simulink model "cst_planning"  (R2023a)
settings: configuration reference "config" (kept outside this file)
undefined symbols (not defined in the file): DiscIntNeverNeededParam
settings Model: DataDictionary=model_config.sldd  Creator=huangcheng  LastModifiedBy=Administrator
settings ConfigSetRef: SourceName=config

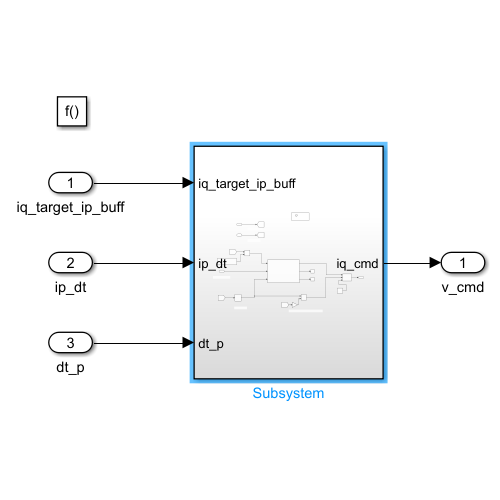
[thumbnail: Simulink's stored preview of the top-level diagram]
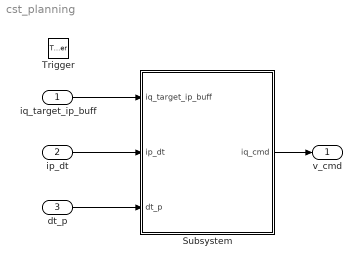
== system cst_planning ==
  iq_target_ip_buff : Inport  OutDataTypeStr=single  PortDimensions=4
  ip_dt : Inport  Port=2
  dt_p : Inport  Port=3
  Trigger : TriggerPort  TriggerType=function-call  VariantControl=(inherit)  PortDimensions=1
  Subsystem : Subsystem
  v_cmd : Outport
  wires:
  iq_target_ip_buff/1 -> Subsystem/1(iq_target_ip_buff)
  ip_dt/1 -> Subsystem/2(ip_dt)
  Subsystem/1(iq_cmd) -> v_cmd/1
  dt_p/1 -> Subsystem/3(dt_p)

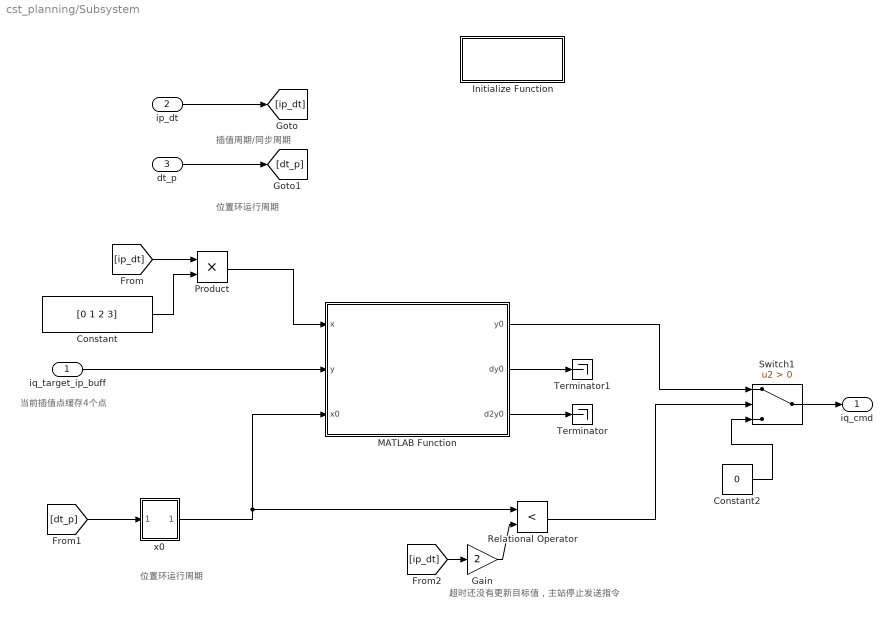
== system cst_planning/Subsystem ==
  note: 插值周期/同步周期
  note: 位置环运行周期
  note: 当前插值点缓存4个点
  note: 位置环运行周期
  note: 超时还没有更新目标值，主站停止发送指令
  iq_target_ip_buff : Inport  OutDataTypeStr=single  PortDimensions=4
  ip_dt : Inport  Port=2
  dt_p : Inport  Port=3
  Constant : Constant  Value=[0 1 2 3]  OutDataTypeStr=single
  Constant2 : Constant  Value=0  OutDataTypeStr=single
  Gain : Gain  Gain=2
  Initialize Function : Subsystem  TreatAsAtomicUnit=on
  MATLAB Function : MATLAB Function  SystemSampleTime=10e-5
  Product : Product
  Relational Operator : RelationalOperator  Operator=<  OutDataTypeStr=boolean  RndMeth=Simplest  InputSameDT=off
  Switch1 : Switch  Criteria=u2 > Threshold  SaturateOnIntegerOverflow=off  InputSameDT=off
  Terminator : Terminator
  Terminator1 : Terminator
  x0 : Subsystem
  iq_cmd : Outport
  wires:
  dt_p/1 -> [dt_p]
  ip_dt/1 -> [ip_dt]
  iq_target_ip_buff/1 -> MATLAB Function/2(y)
  Constant/1 -> Product/2
  MATLAB Function/3(d2y0) -> Terminator/1
  Product/1 -> MATLAB Function/1(x)
  [ip_dt] -> Product/1
  MATLAB Function/2(dy0) -> Terminator1/1
  [dt_p] -> x0/1(In1)
  [ip_dt] -> Gain/1
  Gain/1 -> Relational Operator/2
  Relational Operator/1 -> Switch1/2
  x0/1(x0) -> Relational Operator/1, MATLAB Function/3(x0)
  Constant2/1 -> Switch1/3
  Switch1/1 -> iq_cmd/1
  MATLAB Function/1(y0) -> Switch1/1

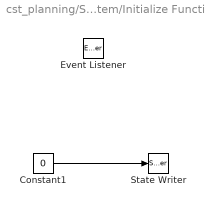
== system cst_planning/Subsystem/Initialize Function ==
  Constant1 : Constant  Value=0  OutDataTypeStr=single
  Event Listener : EventListener  DisableCoverage=on  EventName=reset
  State Writer : StateWriter  StateOwnerBlock=../../x0/Discrete-Time Integrator  StateName=x0_sum
  wires:
  Constant1/1 -> State Writer/1

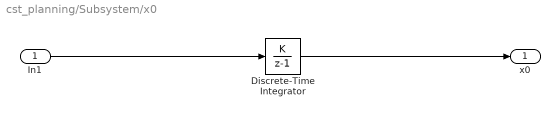
== system cst_planning/Subsystem/x0 ==
  In1 : Inport
  Discrete-Time Integrator : DiscreteIntegrator  IntegratorMethod=Accumulation: Forward Euler  SampleTime=-1  StateName=x0_sum  ICPrevOutput=DiscIntNeverNeededParam  ICPrevScaledInput=DiscIntNeverNeededParam
  x0 : Outport
  wires:
  In1/1 -> Discrete-Time Integrator/1
  Discrete-Time Integrator/1 -> x0/1

== matlab function cst_planning/Subsystem/MATLAB Function ==
  data: x input; y input; y0 output; x0 input; dy0 output; d2y0 output
function [y0, dy0, d2y0]  = InterpolateSignal(x,y,x0)
 
 % 可选插值方法pchip、 makima 、spline一阶导数和二阶导数
    % 输入:
    %   pp - 返回的分段多项式结构
    %   x0 - 要计算的点（可以是向量）
    % 输出:
    %   y0  - 函数值
    %   dy0 - 一阶导数
    %   d2y0 - 二阶导数

    % 提取分段插值起点, 插值计算都减去起点
    y_init = y(1);
    yy = y - y_init;

    pp = makima(x, yy);


    % 1. 计算函数值
    y0 = ppval(pp, x0) + y_init;
    
     % 方法二：手动从系数计算
    breaks = pp.breaks;
    coefs = pp.coefs;

    %x0必须始终在插值第一段
 
    c = coefs(1, :);  % 系数为 [a, b, c, d]，对应 (x-break)^3, (x-break)^2, (x-break)^1, 常数项
    t = x0 - breaks(1);
    % 一阶导数
    dy0 = 3*c(1)*t^2 + 2*c(2)*t + c(3);
    % 二阶导数
    d2y0 = 6*c(1)*t + 2*c(2);

end
